simulink model "pack_sim"  (R2025a)
settings: Solver=FixedStepDiscrete  StartTime=0.0  StopTime=nLaps*T_lap  FixedStep=dt  RelTol=1e-3
values from neighbouring files (symbols this model uses):
  dt = 0.02    [pack_profile.mat]
  I_max = 100    [pack_profile.mat]    (also in report.m = 104)
  P_cap = 22890    [pack_profile.mat]
  V0_pack = 470.4    [pack_profile.mat]
  Vc_min = 2.5    [pack_profile.mat]
libraries: simulink x1, Molicel_INR18650P28A_241c01110_lib x1
settings Model: Creator=akevi  LastModifiedBy=akevi

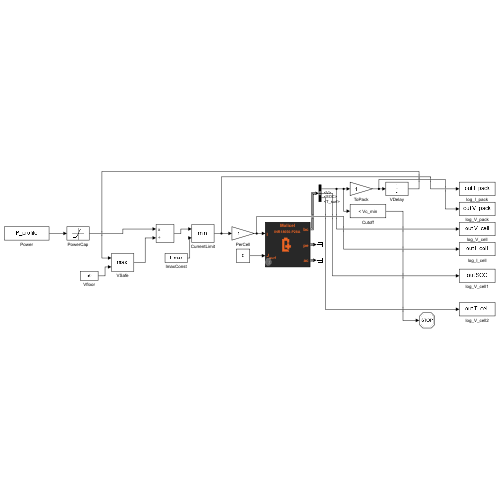
[thumbnail: Simulink's stored preview of the top-level diagram]
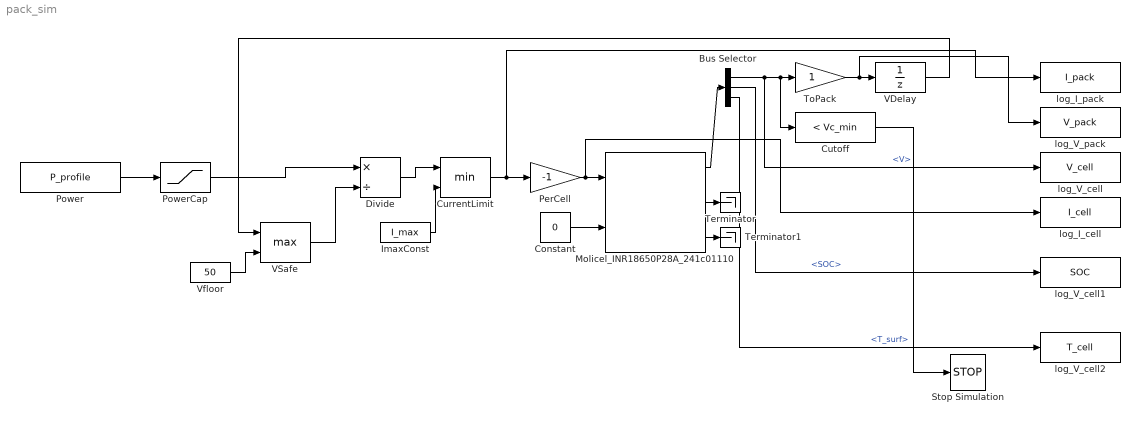
== system pack_sim ==
  Bus Selector : BusSelector  OutputSignals=V,SOC,T_surf
  Constant : Constant  Value=0
  CurrentLimit : MinMax  Inputs=2
  Cutoff : simulink/Logic and Bit Operations/Compare To Constant  relop=<  const=Vc_min  OutDataTypeStr=boolean
  Divide : Product  Inputs=*/
  ImaxConst : Constant  Value=I_max
  Molicel_INR18650P28A_241c01110 : Molicel_INR18650P28A_241c01110_lib/Molicel_INR18650P28A_241c01110  Tag=Molicel_INR18650P28A_241c01110  Description=Batemo Battery Model of a single cell of type BatteryName.  init_start=1  callback_running=0  enable_addon_pe=off  enable_addon_ac=off  enable_addon_ap=off  select_initial_SOC_OCV=SOC  select_initial_charge_discharge=Charge  SOC_0=100.0  V_ocv_0=3.35  T_inner_0=25  N_serial=112  N_parallel=5  select_input_I_V=Current Input  select_input_J_T=Heat Current Input  k_C_fu=100  k_loss_fu=100  select_aging_mode=Operating Point  select_evolution=none  select_extrapolation_method=Linear  select_accuracylevel=Standard  select_aging_scenario=Standard  select_aging_scenario_internal=Standard  SOH_C=100  SOH_R=100  k_C_an=100  k_C_ca=100  k_C_li=100  k_C_an1=100  k_C_ca1=100  k_C_x=100  k_loss_short=100  k_loss_medium=100  k_loss_long=100  SOH_C_expert=100  SOH_R_expert=100  x_evolution=0  unit_evolution=Time under Test  SOH_C_evolution=100  k_C_an_evolution=100  k_C_ca_evolution=100  k_C_li_evolution=100  k_C_an1_evolution=100  k_C_ca1_evolution=100  k_C_x_evolution=100  SOH_R_evolution=100  k_loss_short_evolution=100  k_loss_medium_evolution=100  k_loss_long_evolution=100  select_accuracylevel_evolution=Standard  x_evolutioninterpolation1=100  x_evolutioninterpolation2=100  x_evolutioninterpolation3=100  evolutions_path=C:/Program Files/Batemo Cell Model Custom/R2025a/Molicel_INR18650P28A_241c01110/evolutions  enable_addon_lbc=off  enable_addon_lpe=off  enable_addon_lac=off  tau_filter=1e-07  T_inner_feedthrough=off  SOC_def_enable=0  SOC_def_1=4.2  SOC_def_2=2e4  show_all_aging_scenarios=off  init_stop=0
  PerCell : Gain  Gain=-1
  Power : FromWorkspace  VariableName=P_profile  SampleTime=dt  OutputAfterFinalValue=Holding final value
  PowerCap : Saturate  UpperLimit=P_cap  LowerLimit=0
  Stop Simulation : Stop
  Terminator : Terminator
  Terminator1 : Terminator
  ToPack : Gain
  VDelay : UnitDelay  InitialCondition=V0_pack  SampleTime=dt  HasFrameUpgradeWarning=on
  VSafe : MinMax  Function=max  Inputs=2
  Vfloor : Constant  Value=50
  log_I_cell : ToWorkspace  VariableName=I_cell  SaveFormat=Timeseries  SampleTime=-1
  log_I_pack : ToWorkspace  VariableName=I_pack  SaveFormat=Timeseries  SampleTime=-1
  log_V_cell : ToWorkspace  VariableName=V_cell  SaveFormat=Timeseries  SampleTime=-1
  log_V_cell1 : ToWorkspace  VariableName=SOC  SaveFormat=Timeseries  SampleTime=-1
  log_V_cell2 : ToWorkspace  VariableName=T_cell  SaveFormat=Timeseries  SampleTime=-1
  log_V_pack : ToWorkspace  VariableName=V_pack  SaveFormat=Timeseries  SampleTime=-1
  wires:
  PerCell/1 -> log_I_cell/1, Molicel_INR18650P28A_241c01110/1
  Power/1 -> PowerCap/1
  PowerCap/1 -> Divide/1
  Vfloor/1 -> VSafe/2
  VSafe/1 -> Divide/2
  ImaxConst/1 -> CurrentLimit/2
  Divide/1 -> CurrentLimit/1
  CurrentLimit/1 -> log_I_pack/1, PerCell/1
  Constant/1 -> Molicel_INR18650P28A_241c01110/2
  Molicel_INR18650P28A_241c01110/1 -> Bus Selector/1
  Bus Selector/1 -> log_V_cell/1, Cutoff/1, ToPack/1  "<V>"
  ToPack/1 -> log_V_pack/1, VDelay/1
  VDelay/1 -> VSafe/1
  Cutoff/1 -> Stop Simulation/1
  Bus Selector/2 -> log_V_cell1/1  "<SOC>"
  Bus Selector/3 -> log_V_cell2/1  "<T_surf>"
  Molicel_INR18650P28A_241c01110/2 -> Terminator/1
  Molicel_INR18650P28A_241c01110/3 -> Terminator1/1
